simulink model "hovorka_artificial_pancreas"  (R2024a)
settings: Solver=ode15s  StartTime=0.0  StopTime=720  RelTol=1e-6  AbsTol=1e-8
InitFcn:
  | addpath(fullfile(fileparts(which('hovorka_artificial_pancreas')), '..', 'scripts')); p = hovorka_params(70, 100); [mpc_obj, plant_ss_d] = design_mpc_controller();
libraries: mpclib x1
settings Model: Creator=drkod  LastModifiedBy=drkod

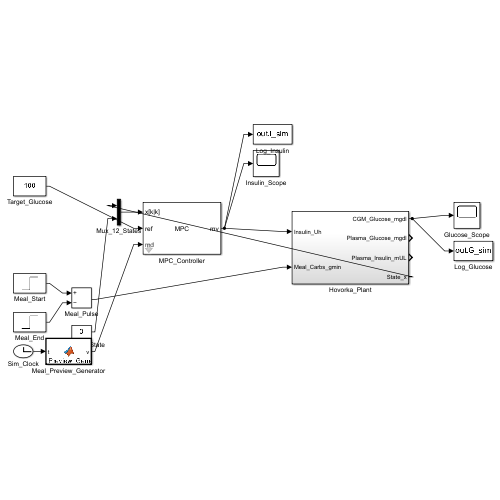
[thumbnail: Simulink's stored preview of the top-level diagram]
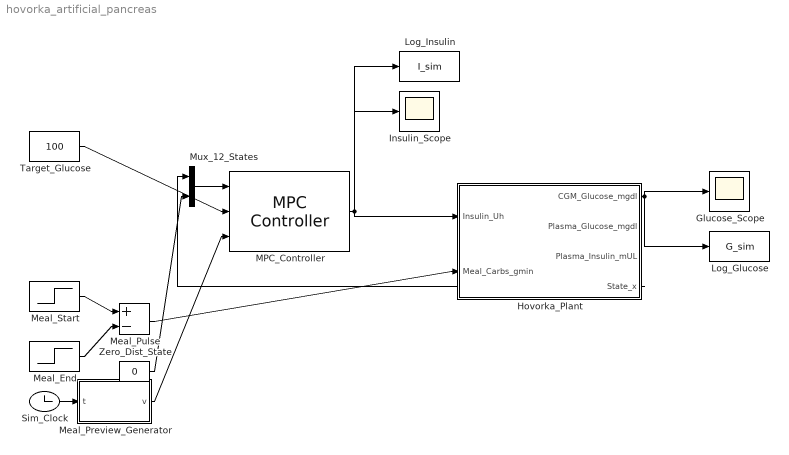
== system hovorka_artificial_pancreas ==
  Glucose_Scope : Scope
  Hovorka_Plant : Subsystem
  Insulin_Scope : Scope
  Log_Glucose : ToWorkspace  VariableName=G_sim  SaveFormat=Timeseries  SampleTime=-1
  Log_Insulin : ToWorkspace  VariableName=I_sim  SaveFormat=Timeseries  SampleTime=-1
  MPC_Controller : mpclib/MPC Controller  SCDEnableBlockLinearizationSpecification=on  mpcobj=mpc_obj  is_multiple=0  enable_value=0  return_u0=off  updateMPCinCallerWorkspace=on  md_inport=on  mv_inport=off  uref_inport=off  return_cost=off  return_mvseq=off  return_qpstatus=off  return_xseq=off  return_state=off  return_ovseq=off  state_inport=on  umin_inport=off  umax_inport=off  ymin_inport=off  ymax_inport=off  cc_inport=off  ywt_inport=off  uwt_inport=off  duwt_inport=off  rhoeps_inport=off  pm_inport=off  MaximumP=10  HorizonChoice=FixedHorizon  n_ts=1  n_p=10  n_mv=1  n_md=1  n_ud=0  n_mo=1  n_uo=0  BlockDataType=double  SampleTimeInherited=off  switch_inport=off
  Meal_End : Step  Time=135  After=3.3333  SampleTime=0
  Meal_Preview_Generator : MATLAB Function  TreatAsAtomicUnit=on
  Meal_Pulse : Sum  Inputs=+-
  Meal_Start : Step  Time=120  After=3.3333  SampleTime=0
  Mux_12_States : Mux  Inputs=2
  Sim_Clock : Clock
  Target_Glucose : Constant  Value=100
  Zero_Dist_State : Constant  Value=0
  wires:
  Meal_Start/1 -> Meal_Pulse/1
  Meal_End/1 -> Meal_Pulse/2
  Sim_Clock/1 -> Meal_Preview_Generator/1(t)
  Hovorka_Plant/4(State_x) -> Mux_12_States/1
  Zero_Dist_State/1 -> Mux_12_States/2
  Mux_12_States/1 -> MPC_Controller/1
  Target_Glucose/1 -> MPC_Controller/2
  Meal_Preview_Generator/1(v) -> MPC_Controller/3
  MPC_Controller/1 -> Hovorka_Plant/1(Insulin_Uh), Insulin_Scope/1, Log_Insulin/1
  Meal_Pulse/1 -> Hovorka_Plant/2(Meal_Carbs_gmin)
  Hovorka_Plant/1(CGM_Glucose_mgdl) -> Glucose_Scope/1, Log_Glucose/1

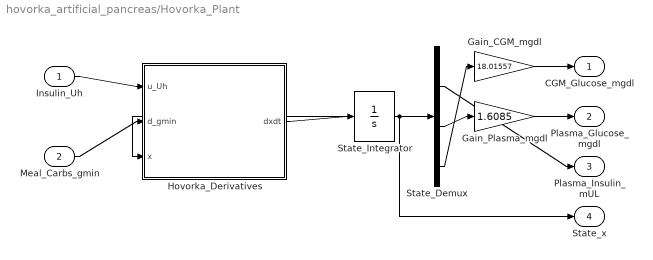
== system hovorka_artificial_pancreas/Hovorka_Plant ==
  Insulin_Uh : Inport
  Meal_Carbs_gmin : Inport  Port=2
  Gain_CGM_mgdl : Gain  Gain=18.01557
  Gain_Plasma_mgdl : Gain  Gain=1.6085
  Hovorka_Derivatives : MATLAB Function  TreatAsAtomicUnit=on
  State_Demux : Demux  Outputs=11
  State_Integrator : Integrator  InitialCondition=p.ss.x0
  CGM_Glucose_mgdl : Outport
  Plasma_Glucose_mgdl : Outport  Port=2
  Plasma_Insulin_mUL : Outport  Port=3
  State_x : Outport  Port=4
  wires:
  Insulin_Uh/1 -> Hovorka_Derivatives/1(u_Uh)
  Meal_Carbs_gmin/1 -> Hovorka_Derivatives/2(d_gmin)
  State_Integrator/1 -> Hovorka_Derivatives/3(x), State_Demux/1, State_x/1
  Hovorka_Derivatives/1(dxdt) -> State_Integrator/1
  State_Demux/11 -> Gain_CGM_mgdl/1
  State_Demux/7 -> Gain_Plasma_mgdl/1
  Gain_CGM_mgdl/1 -> CGM_Glucose_mgdl/1
  Gain_Plasma_mgdl/1 -> Plasma_Glucose_mgdl/1
  State_Demux/3 -> Plasma_Insulin_mUL/1

== matlab function hovorka_artificial_pancreas/Meal_Preview_Generator ==
  data: t input; v output
function v = Meal_Preview_Generator(t)
% Meal preview lookahead over prediction horizon (49 steps)
v = zeros(49, 1);
for h = 0:48
    tf = t + h * 5.0;
    if tf >= 120.0 && tf < 135.0
        v(h + 1) = 3.3333;
    end
end
end

== matlab function hovorka_artificial_pancreas/Hovorka_Plant/Hovorka_Derivatives ==
  data: u_Uh input; dxdt output; d_gmin input; x input
function dxdt = Hovorka_Derivatives(u_Uh, d_gmin, x)
%#codegen
BW = 70.0; V_G = 0.16 * BW; V_I = 0.12 * BW; k12 = 0.066;
F01 = 0.0097 * BW; EGP0 = 0.0161 * BW; ke = 0.138; tau_S = 55.0; tau_D = 40.0; A_G = 0.80; tau_cgm = 10.0;
ka1 = 0.006; ka2 = 0.06; ka3 = 0.03; kb1 = ka1 * 51.2e-4; kb2 = ka2 * 8.2e-4; kb3 = ka3 * 520e-4;
u_mumin = u_Uh * (1000.0 / 60.0); d_mmolmin = d_gmin * (1000.0 / 180.1557);
S1 = max(0.0, x(1)); S2 = max(0.0, x(2)); I = max(0.0, x(3));
x1 = max(0.0, x(4)); x2 = max(0.0, x(5)); x3 = max(0.0, x(6));
Q1 = max(0.01, x(7)); Q2 = max(0.01, x(8)); D1 = max(0.0, x(9)); D2 = max(0.0, x(10)); G_meas = max(0.01, x(11));
UI = S2 / tau_S; dS1 = u_mumin - S1 / tau_S; dS2 = (S1 - S2) / tau_S;
dI = UI / V_I - ke * I;
dx1 = -ka1 * x1 + kb1 * I; dx2 = -ka2 * x2 + kb2 * I; dx3 = -ka3 * x3 + kb3 * I;
UG = D2 / tau_D; dD1 = d_mmolmin * A_G - D1 / tau_D; dD2 = (D1 - D2) / tau_D;
G = Q1 / V_G;
if G >= 4.5, F01_c = F01; else, F01_c = F01 * (G / 4.5); end
if G >= 9.0, FR = 0.003 * (G - 9.0) * V_G; else, FR = 0.0; end
EGP = max(0.0, EGP0 * (1.0 - x3));
dQ1 = -(F01_c + x1 * Q1) + k12 * Q2 - FR + EGP + UG;
dQ2 = x1 * Q1 - (k12 + x2) * Q2;
dG_meas = (G - G_meas) / tau_cgm;
dxdt = [dS1; dS2; dI; dx1; dx2; dx3; dQ1; dQ2; dD1; dD2; dG_meas];
end
